simulink model "grid_foll_vsc"  (R2024b)
settings: Solver=ode5  StartTime=0.0  StopTime=t_sim  FixedStep=T_sim  MaxStep=1e-4  RelTol=1e-5
values from neighbouring files (symbols this model uses):
  ext = 1    [init_and_run_perturbed_case.m]
  L_f1 = 0.08*l_b    (= 0.024514105368)    [init_and_run_perturbed_case.m]
  params = [w_b, L_f1, L_f2, tau_pll, K_pll, tau_i, K_i]    [init_and_run_perturbed_case.m]    (also in init_emt2.m = [w_b, l_f, kp_i, ki_i, kp_pll_f, ki_pll_f, kp_pll, ki_pll])
  r_f1 = 0.1*L_f1*w_b    (= 0.770133333333)    [init_and_run_perturbed_case.m]
  T_sample = 2e-4    (= 0.0002)    [init_and_run_perturbed_case.m]    (also in init_emt2.m)
  T_sim = 1e-6    (= 1e-06)    [init_and_run_perturbed_case.m]    (also in init_emt2.m)
libraries: spsControlledVoltageSourceLib x6, spsGroundLib x2, spsThreePhaseSeriesRLCBranchLib x1, spsThreePhaseVIMeasurementLib x1, sps_lib x1
settings Model: Creator=carlo  LastModifiedBy=carlo
settings DataIOCC: ReturnWorkspaceOutputs=off

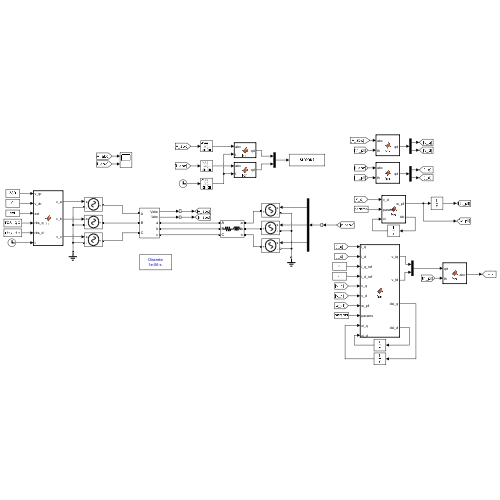
[thumbnail: Simulink's stored preview of the top-level diagram]
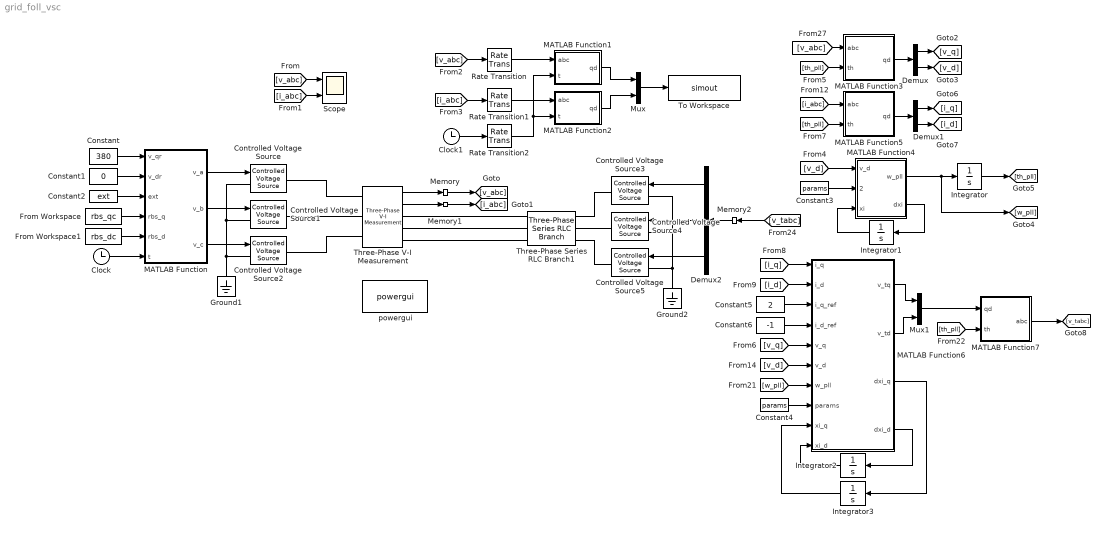
== system grid_foll_vsc ==
  Clock : Clock
  Clock1 : Clock
  Constant : Constant  Value=380
  Constant1 : Constant  Value=0
  Constant2 : Constant  Value=ext
  Constant3 : Constant  Value=params
  Constant4 : Constant  Value=params
  Constant5 : Constant  Value=2
  Constant6 : Constant  Value=-1
  Controlled Voltage Source{,1..5} (6 alike) : spsControlledVoltageSourceLib/Controlled Voltage Source  Initialize=on  Source_Type=AC  Amplitude=0  Phase=0  Frequency=0  Measurements=None
  Demux : Demux  Outputs=2
  Demux1 : Demux  Outputs=2
  Demux2 : Demux  Outputs=3
  From Workspace : FromWorkspace  VariableName=rbs_qc  SampleTime=T_sample
  From Workspace1 : FromWorkspace  VariableName=rbs_dc  SampleTime=T_sample
  Ground1 : spsGroundLib/Ground  LConnTagsString=a
  Ground2 : spsGroundLib/Ground  LConnTagsString=a
  Integrator{,1..3} (4 alike) : Integrator
  MATLAB Function : MATLAB Function  TreatAsAtomicUnit=on
  MATLAB Function1 : MATLAB Function  TreatAsAtomicUnit=on
  MATLAB Function2 : MATLAB Function  TreatAsAtomicUnit=on
  MATLAB Function3 : MATLAB Function  TreatAsAtomicUnit=on
  MATLAB Function4 : MATLAB Function  TreatAsAtomicUnit=on
  MATLAB Function5 : MATLAB Function  TreatAsAtomicUnit=on
  MATLAB Function6 : MATLAB Function  TreatAsAtomicUnit=on
  MATLAB Function7 : MATLAB Function  TreatAsAtomicUnit=on
  Memory : Memory
  Memory1 : Memory
  Memory2 : Memory
  Mux : Mux  Inputs=2
  Mux1 : Mux  Inputs=2
  Rate Transition : RateTransition  OutPortSampleTime=T_sample
  Rate Transition1 : RateTransition  OutPortSampleTime=T_sample
  Rate Transition2 : RateTransition  OutPortSampleTime=T_sample
  Scope : Scope  NumInputPorts=2
  Three-Phase Series RLC Branch1 : spsThreePhaseSeriesRLCBranchLib/Three-Phase Series RLC Branch  LConnTagsString=A|B|C  RConnTagsString=A|B|C  BranchType=RL  Resistance=r_f1  Inductance=L_f1  Capacitance=1e-6  Measurements=None
  Three-Phase V-I Measurement : spsThreePhaseVIMeasurementLib/Three-Phase V-I Measurement  VoltageMeasurement=phase-to-ground  SetLabelV=off  LabelV=Vabc  Vpu=off  VpuLL=off  CurrentMeasurement=yes  SetLabelI=off  LabelI=Iabc  Ipu=off  Pbase=100e6  Vbase=500e3  OutputType=Complex  PhasorSimulation=off  PSBequivalent=0
  To Workspace : ToWorkspace  VariableName=simout  SaveFormat=Timeseries  SampleTime=-1
  powergui : sps_lib/powergui  Priority=1  SimulationMode=Discrete  SampleTime=T_sim  frequency=60  Iterations=50  frequencyindice=0  Pbase=100e6  ErrMax=1e-4  UnitsV=kV  UnitsW=MW  buscounter=0  FunctionMessages=off  echomessages=off  EnableUseOfTLC=off  CurrentSourceSwitches=off  DisableSnubberDevices=off  DisableRonSwitches=off  DisableVfSwitches=off  DisplayEquations=off  AutomaticDiscreteSolvers=off  SolverType=Tustin/Backward Euler (TBE)  Interpol=off  ExternalGateDelay=off  methode=off  Ts=100  x0status=blocks  SPID=on  SwTol=0  HookPort=off  NonlinearTolerance=1e-4  nMaxIteration=100  ContinueOnMaxIteration=off  RestoreLinks=warning  ResistiveCurrentMeasurement=off  Frange=[0:2:500]  Ylog=off  Xlog=on  ShowGrid=off  save=off  variable=ZData  structure=0  ZoomFFT=off  StartTime=0.0  cycles=1  DisplayStyle=1  fundamental=60  FreqAxis=off  MaxFrequency=1000  frequencyindicesteady=1  RmsSteady=1  display=off
  wires:
  MATLAB Function/1(v_a) -> Controlled Voltage Source/1
  MATLAB Function/2(v_b) -> Controlled Voltage Source1/1
  MATLAB Function/3(v_c) -> Controlled Voltage Source2/1
  From Workspace1/1 -> MATLAB Function/5(rbs_d)
  From Workspace/1 -> MATLAB Function/4(rbs_q)
  Constant/1 -> MATLAB Function/1(v_qr)
  Constant1/1 -> MATLAB Function/2(v_dr)
  Constant2/1 -> MATLAB Function/3(ext)
  Clock/1 -> MATLAB Function/6(t)
  Three-Phase V-I Measurement/1 -> Memory/1
  Three-Phase V-I Measurement/2 -> Memory1/1
  [v_abc] -> Scope/1
  [i_abc] -> Scope/2
  [v_abc] -> Rate Transition/1
  [i_abc] -> Rate Transition1/1
  Clock1/1 -> Rate Transition2/1
  Rate Transition/1 -> MATLAB Function1/1(abc)
  Rate Transition1/1 -> MATLAB Function2/1(abc)
  Rate Transition2/1 -> MATLAB Function2/2(t), MATLAB Function1/2(t)
  Mux/1 -> To Workspace/1
  MATLAB Function2/1(qd) -> Mux/2
  MATLAB Function1/1(qd) -> Mux/1
  MATLAB Function5/1(qd) -> Demux1/1
  [v_d] -> MATLAB Function6/6(v_d)
  Constant6/1 -> MATLAB Function6/4(i_d_ref)
  Demux/1 -> [v_q]
  Demux1/1 -> [i_q]
  [i_q] -> MATLAB Function6/1(i_q)
  [i_abc] -> MATLAB Function5/1(abc)
  MATLAB Function4/1(w_pll) -> [w_pll], Integrator/1
  MATLAB Function6/2(v_td) -> Mux1/2
  [th_pll] -> MATLAB Function7/2(th)
  [i_d] -> MATLAB Function6/2(i_d)
  Constant4/1 -> MATLAB Function6/8(params)
  [v_d] -> MATLAB Function4/1(v_d)
  MATLAB Function3/1(qd) -> Demux/1
  [v_abc] -> MATLAB Function3/1(abc)
  MATLAB Function6/1(v_tq) -> Mux1/1
  Integrator1/1 -> MATLAB Function4/3(xi)
  Constant5/1 -> MATLAB Function6/3(i_q_ref)
  Demux1/2 -> [i_d]
  [th_pll] -> MATLAB Function3/2(th)
  MATLAB Function4/2(dxi) -> Integrator1/1
  [w_pll] -> MATLAB Function6/7(w_pll)
  MATLAB Function6/3(dxi_q) -> Integrator3/1
  [v_q] -> MATLAB Function6/5(v_q)
  Integrator2/1 -> MATLAB Function6/10(xi_d)
  Demux/2 -> [v_d]
  Integrator/1 -> [th_pll]
  Mux1/1 -> MATLAB Function7/1(qd)
  MATLAB Function6/4(dxi_d) -> Integrator2/1
  Integrator3/1 -> MATLAB Function6/9(xi_q)
  [th_pll] -> MATLAB Function5/2(th)
  Constant3/1 -> MATLAB Function4/2(params)
  Memory/1 -> [v_abc]
  Memory1/1 -> [i_abc]
  Demux2/1 -> Controlled Voltage Source3/1
  Demux2/2 -> Controlled Voltage Source4/1
  Demux2/3 -> Controlled Voltage Source5/1
  [v_tabc] -> Memory2/1
  MATLAB Function7/1(abc) -> [v_tabc]
  Memory2/1 -> Demux2/1
  connections:
  Controlled Voltage Source1/RConn1 -- Three-Phase V-I Measurement/LConn2
  Controlled Voltage Source/RConn1 -- Three-Phase V-I Measurement/LConn1
  Controlled Voltage Source2/RConn1 -- Three-Phase V-I Measurement/LConn3
  Ground1/LConn1 -- Controlled Voltage Source2/LConn1 -- Controlled Voltage Source/LConn1 -- Controlled Voltage Source1/LConn1
  Three-Phase Series RLC Branch1/LConn3 -- Three-Phase V-I Measurement/RConn3
  Three-Phase V-I Measurement/RConn1 -- Three-Phase Series RLC Branch1/LConn1
  Three-Phase V-I Measurement/RConn2 -- Three-Phase Series RLC Branch1/LConn2
  Three-Phase Series RLC Branch1/RConn2 -- Controlled Voltage Source4/RConn1
  Three-Phase Series RLC Branch1/RConn1 -- Controlled Voltage Source3/RConn1
  Three-Phase Series RLC Branch1/RConn3 -- Controlled Voltage Source5/RConn1
  Controlled Voltage Source5/LConn1 -- Controlled Voltage Source4/LConn1 -- Controlled Voltage Source3/LConn1 -- Ground2/LConn1

== matlab function grid_foll_vsc/MATLAB Function1 ==
  data: abc input; qd output; t input
function qd = fcn(abc,t)

w = 100*pi;
th = w*t;
d = 2*pi/3;

Tb = [cos(th), cos(th - d), cos(th + d);
     -sin(th),-sin(th - d),-sin(th + d)];

qd = Tb*abc;

== matlab function grid_foll_vsc/MATLAB Function ==
  data: v_qr input; v_a output; v_dr input; ext input; rbs_q input; rbs_d input; t input; v_b output; v_c output
function [v_a, v_b, v_c] = fcn(v_qr, v_dr, ext, rbs_q, rbs_d, t)


v_q = v_qr + ext*rbs_q*120;
v_d = v_dr + ext*rbs_d*120;
w = 100*pi;
th = w*t;
d = 2*pi/3;

Tb = [cos(th),     -sin(th);
      cos(th - d), -sin(th -d);
      cos(th + d), -sin(th+d)];

v_abc = Tb*[v_q; v_d];
v_a = v_abc(1);
v_b = v_abc(2);
v_c = v_abc(3);

== matlab function grid_foll_vsc/MATLAB Function2 ==
  data: abc input; qd output; t input
function qd = fcn(abc,t)

w = 100*pi;
th = w*t;
d = 2*pi/3;

Tb = [cos(th), cos(th - d), cos(th + d);
     -sin(th),-sin(th - d),-sin(th + d)];

qd = Tb*abc;

== matlab function grid_foll_vsc/MATLAB Function3 ==
  data: abc input; qd output; th input
function qd = fcn(abc, th)

Tb = 2/3*[cos(th), cos(th - 2*pi/3), cos(th + 2*pi/3);
         -sin(th),-sin(th - 2*pi/3),-sin(th + 2*pi/3)];
qd = Tb*abc;

== matlab function grid_foll_vsc/MATLAB Function4 ==
  data: v_d input; w_pll output; params input; xi input; dxi output
function [w_pll, dxi] = fcn(v_d, params, xi)

w_ref = params(1);
k_pll = params(5);
t_pll = params(4);

err = v_d;
w_pll = k_pll*err + xi + w_ref;
dxi = k_pll/t_pll*err;

== matlab function grid_foll_vsc/MATLAB Function5 ==
  data: abc input; qd output; th input
function qd = fcn(abc, th)

Tb = 2/3*[cos(th), cos(th - 2*pi/3), cos(th + 2*pi/3);
         -sin(th),-sin(th - 2*pi/3),-sin(th + 2*pi/3)];
qd = Tb*abc;

== matlab function grid_foll_vsc/MATLAB Function6 ==
  data: i_q input; i_d input; i_q_ref input; i_d_ref input; v_q input; v_d input; w_pll input; v_tq output; params input; v_td output; xi_q input; xi_d input; dxi_q output; dxi_d output
function [v_tq, v_td, dxi_q, dxi_d] = fcn(i_q, i_d, i_q_ref, i_d_ref, v_q, v_d, w_pll, params, xi_q, xi_d)

l = params(2);
t_i = params(6);
k_i = params(7);

e_q = i_q_ref - i_q;
e_d = i_d_ref - i_d;

u_tq = k_i*e_q + xi_q;
u_td = k_i*e_d + xi_d;

v_tq = -u_tq - w_pll*l*i_d - v_q;
v_td = -u_td + w_pll*l*i_q - v_d;

dxi_q = k_i/t_i*e_q;
dxi_d = k_i/t_i*e_d;

== matlab function grid_foll_vsc/MATLAB Function7 ==
  data: qd input; abc output; th input
function abc = fcn(qd, th)

Tb = [cos(th),-sin(th);
      cos(th - 2*pi/3),-sin(th - 2*pi/3);
      cos(th + 2*pi/3),-sin(th + 2*pi/3)];
abc = Tb*qd;
